simulink model "V_Kaynak_QC_Robot"  (R2026b)
settings: Solver=ode4  StopTime=650  FixedStep=0.01
libraries: simulink x2
settings Model: Creator=Dikme  LastModifiedBy=Dikme

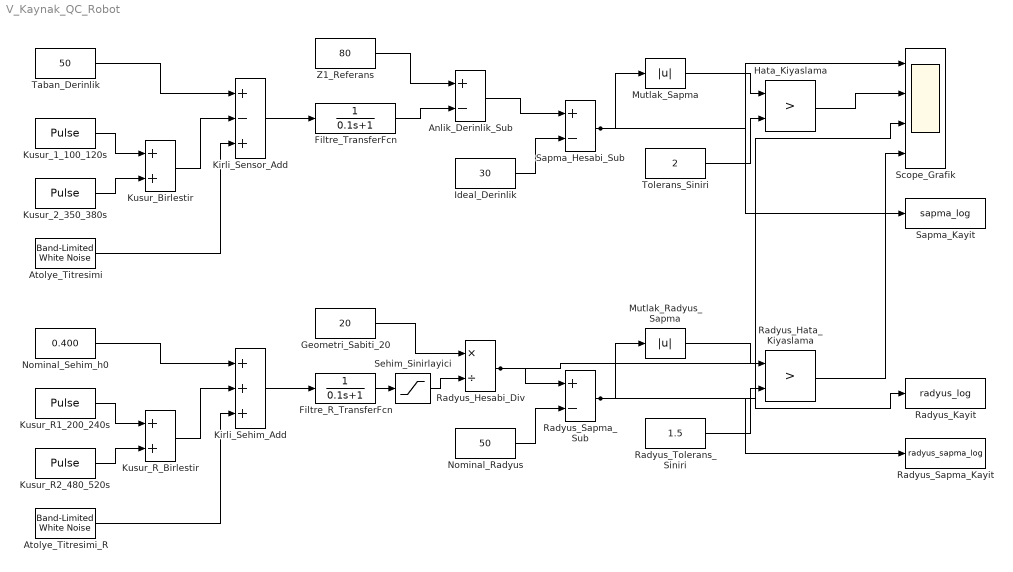
== system V_Kaynak_QC_Robot ==
  Anlik_Derinlik_Sub : Sum  Inputs=+-
  Atolye_Titresimi : simulink/Sources/Band-Limited White Noise  Cov=0.001  Ts=0.01  seed=[23341]
  Atolye_Titresimi_R : simulink/Sources/Band-Limited White Noise  Cov=0.0001  Ts=0.01  seed=[54321]
  Filtre_R_TransferFcn : TransferFcn  Denominator=[0.1 1]
  Filtre_TransferFcn : TransferFcn  Denominator=[0.1 1]
  Geometri_Sabiti_20 : Constant  Value=20
  Hata_Kiyaslama : RelationalOperator  Operator=>  OutDataTypeStr=boolean  RndMeth=Simplest  InputSameDT=off
  Ideal_Derinlik : Constant  Value=30
  Kirli_Sehim_Add : Sum  Inputs=+++
  Kirli_Sensor_Add : Sum  Inputs=+-+
  Kusur_1_100_120s : DiscretePulseGenerator  PulseType=Time based  Amplitude=3.5  Period=1000  PulseWidth=2  PhaseDelay=100
  Kusur_2_350_380s : DiscretePulseGenerator  PulseType=Time based  Amplitude=3.5  Period=1000  PulseWidth=3  PhaseDelay=350
  Kusur_Birlestir : Sum
  Kusur_R1_200_240s : DiscretePulseGenerator  PulseType=Time based  Amplitude=0.1263  Period=1000  PulseWidth=4  PhaseDelay=200
  Kusur_R2_480_520s : DiscretePulseGenerator  PulseType=Time based  Amplitude=-0.0923  Period=1000  PulseWidth=4  PhaseDelay=480
  Kusur_R_Birlestir : Sum
  Mutlak_Radyus_Sapma : Abs  SaturateOnIntegerOverflow=off
  Mutlak_Sapma : Abs  SaturateOnIntegerOverflow=off
  Nominal_Radyus : Constant  Value=50
  Nominal_Sehim_h0 : Constant  Value=0.400
  Radyus_Hata_Kiyaslama : RelationalOperator  Operator=>  OutDataTypeStr=boolean  RndMeth=Simplest  InputSameDT=off
  Radyus_Hesabi_Div : Product  Inputs=*/
  Radyus_Kayit : ToWorkspace  VariableName=radyus_log  SaveFormat=Timeseries  SampleTime=-1
  Radyus_Sapma_Kayit : ToWorkspace  VariableName=radyus_sapma_log  SaveFormat=Timeseries  SampleTime=-1
  Radyus_Sapma_Sub : Sum  Inputs=+-
  Radyus_Tolerans_Siniri : Constant  Value=1.5
  Sapma_Hesabi_Sub : Sum  Inputs=+-
  Sapma_Kayit : ToWorkspace  VariableName=sapma_log  SaveFormat=Timeseries  SampleTime=-1
  Scope_Grafik : Scope  NumInputPorts=4
  Sehim_Sinirlayici : Saturate  UpperLimit=5.0  LowerLimit=0.05
  Taban_Derinlik : Constant  Value=50
  Tolerans_Siniri : Constant  Value=2
  Z1_Referans : Constant  Value=80
  wires:
  Kusur_1_100_120s/1 -> Kusur_Birlestir/1
  Kusur_2_350_380s/1 -> Kusur_Birlestir/2
  Taban_Derinlik/1 -> Kirli_Sensor_Add/1
  Kusur_Birlestir/1 -> Kirli_Sensor_Add/2
  Atolye_Titresimi/1 -> Kirli_Sensor_Add/3
  Kirli_Sensor_Add/1 -> Filtre_TransferFcn/1
  Z1_Referans/1 -> Anlik_Derinlik_Sub/1
  Filtre_TransferFcn/1 -> Anlik_Derinlik_Sub/2
  Anlik_Derinlik_Sub/1 -> Sapma_Hesabi_Sub/1
  Ideal_Derinlik/1 -> Sapma_Hesabi_Sub/2
  Sapma_Hesabi_Sub/1 -> Scope_Grafik/1, Sapma_Kayit/1, Mutlak_Sapma/1
  Mutlak_Sapma/1 -> Hata_Kiyaslama/1
  Tolerans_Siniri/1 -> Hata_Kiyaslama/2
  Hata_Kiyaslama/1 -> Scope_Grafik/2
  Kusur_R1_200_240s/1 -> Kusur_R_Birlestir/1
  Kusur_R2_480_520s/1 -> Kusur_R_Birlestir/2
  Nominal_Sehim_h0/1 -> Kirli_Sehim_Add/1
  Kusur_R_Birlestir/1 -> Kirli_Sehim_Add/2
  Atolye_Titresimi_R/1 -> Kirli_Sehim_Add/3
  Kirli_Sehim_Add/1 -> Filtre_R_TransferFcn/1
  Filtre_R_TransferFcn/1 -> Sehim_Sinirlayici/1
  Geometri_Sabiti_20/1 -> Radyus_Hesabi_Div/1
  Sehim_Sinirlayici/1 -> Radyus_Hesabi_Div/2
  Radyus_Hesabi_Div/1 -> Radyus_Kayit/1, Radyus_Sapma_Sub/1
  Nominal_Radyus/1 -> Radyus_Sapma_Sub/2
  Radyus_Sapma_Sub/1 -> Scope_Grafik/3, Radyus_Sapma_Kayit/1, Mutlak_Radyus_Sapma/1
  Mutlak_Radyus_Sapma/1 -> Radyus_Hata_Kiyaslama/1
  Radyus_Tolerans_Siniri/1 -> Radyus_Hata_Kiyaslama/2
  Radyus_Hata_Kiyaslama/1 -> Scope_Grafik/4
